simulink model "StopTrigger_Bench_2"  (R2025b)
settings: Solver=ode23t  StartTime=0.0  StopTime=3  MaxStep=1e-4  RelTol=1e-3
model workspace (MAT data in the model file):
  Ald = 5743.49177499
  GLDR = 1.5
  GPT = 1
  Ipk = 4.37e-06
  R1 = 10000
  Rfix = 10000
  Rhyst = 47000
  Rin = 1000
  Tend = 0.1
  Tstart = 1
  Ttrip = 0.5
  Vcc = 5
  VrefL = 3.82978723404
  VrefP = 2.9375
  gam = 0.8
  seedN = 1
  sigN = 0.01
  t0 = 1
  tau = 0.25
  tauL = 0.05
libraries: fl_lib x68, nesl_utility x24, ee_lib x11, simulink x5
(part 1 of 2)
settings Model: Creator=davin  LastModifiedBy=davin
settings DataIOCC: SaveOutput=off  ReturnWorkspaceOutputs=off

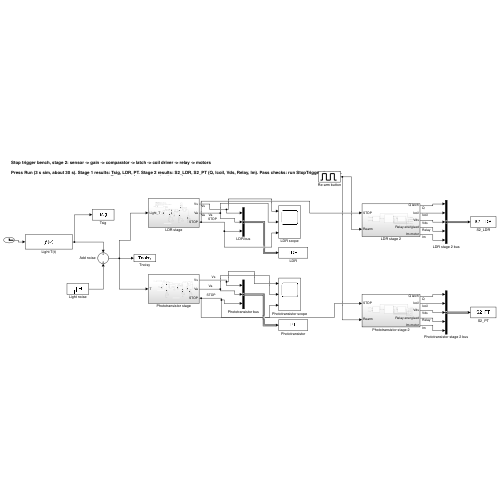
[thumbnail: Simulink's stored preview of the top-level diagram]
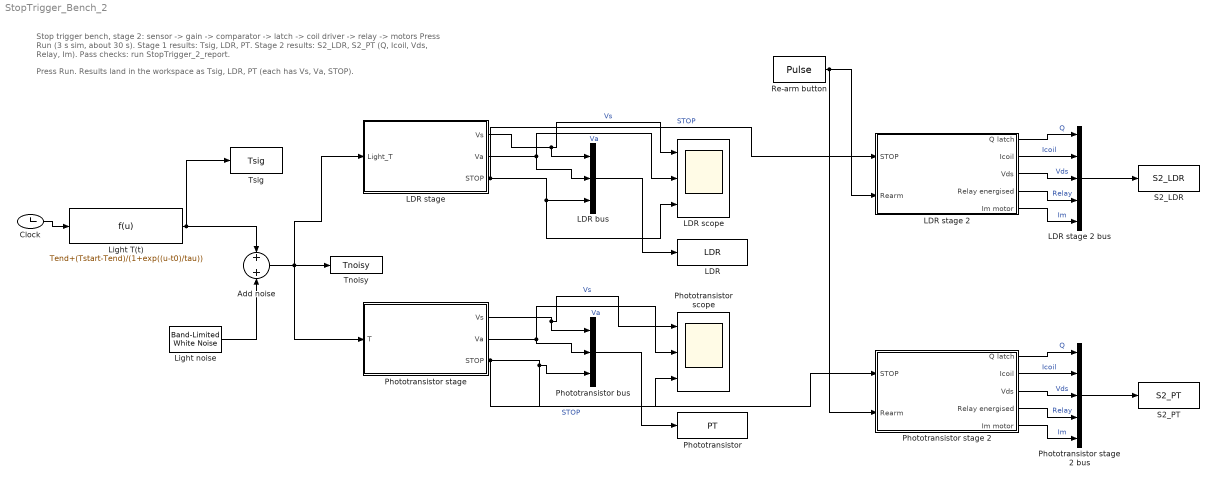
== system StopTrigger_Bench_2 ==
  note: Stop trigger bench, stage 2: sensor -> gain -> comparator -> latch -> coil driver -> relay -> motors
      |
      | Press Run (3 s sim, about 30 s). Stage 1 results: Tsig, LDR, PT. Stage 2 results: S2_LDR, S2_PT (Q, Icoil, Vds, Relay, Im). Pass checks: run StopTrigger_2_report.
  note: Press Run. Results land in the workspace as Tsig, LDR, PT (each has Vs, Va, STOP).
  Add noise : Sum
  Clock : Clock
  LDR : ToWorkspace  VariableName=LDR  SaveFormat=Timeseries  SampleTime=-1
  LDR bus : BusCreator  Inputs=3
  LDR scope : Scope  NumInputPorts=3
      settings: Title=Sensor node Vs (falls when dark)  ActiveDisplayYMinimum=0  ActiveDisplayYMaximum=5  YLabel=Vs [V]
  LDR stage : Subsystem
  LDR stage 2 : Subsystem
  LDR stage 2 bus : BusCreator  Inputs=5
  Light T(t) : Fcn  Expr=Tend+(Tstart-Tend)/(1+exp((u-t0)/tau))
  Light noise : simulink/Sources/Band-Limited White Noise  Cov=sigN^2*0.005  Ts=0.005  seed=[seedN]
  Phototransistor : ToWorkspace  VariableName=PT  SaveFormat=Timeseries  SampleTime=-1
  Phototransistor bus : BusCreator  Inputs=3
  Phototransistor scope : Scope  NumInputPorts=3
      settings: Title=Sensor node Vs (rises when dark)  ActiveDisplayYMinimum=0  ActiveDisplayYMaximum=5  YLabel=Vs [V]
  Phototransistor stage : Subsystem
  Phototransistor stage 2 : Subsystem
  Phototransistor stage 2 bus : BusCreator  Inputs=5
  Re-arm button : DiscretePulseGenerator  PulseType=Time based  Period=2.5  PulseWidth=2  SampleTime=0
  S2_LDR : ToWorkspace  VariableName=S2_LDR  SaveFormat=Timeseries  SampleTime=-1
  S2_PT : ToWorkspace  VariableName=S2_PT  SaveFormat=Timeseries  SampleTime=-1
  Tnoisy : ToWorkspace  VariableName=Tnoisy  SaveFormat=Timeseries  SampleTime=-1
  Tsig : ToWorkspace  VariableName=Tsig  SaveFormat=Timeseries  SampleTime=-1
  wires:
  Clock/1 -> Light T(t)/1
  LDR stage/1(Vs) -> LDR bus/1, LDR scope/1  "Vs"
  LDR stage/2(Va) -> LDR bus/2, LDR scope/2  "Va"
  LDR stage/3(STOP) -> LDR bus/3, LDR scope/3, LDR stage 2/1(STOP)  "STOP"
  LDR bus/1 -> LDR/1
  Phototransistor stage/1(Vs) -> Phototransistor bus/1, Phototransistor scope/1  "Vs"
  Phototransistor stage/2(Va) -> Phototransistor bus/2, Phototransistor scope/2  "Va"
  Phototransistor stage/3(STOP) -> Phototransistor bus/3, Phototransistor scope/3, Phototransistor stage 2/1(STOP)  "STOP"
  Phototransistor bus/1 -> Phototransistor/1
  Light T(t)/1 -> Add noise/1, Tsig/1
  Light noise/1 -> Add noise/2
  Add noise/1 -> LDR stage/1(Light_T), Tnoisy/1, Phototransistor stage/1(T)
  Re-arm button/1 -> LDR stage 2/2(Rearm), Phototransistor stage 2/2(Rearm)
  LDR stage 2/1(Q latch) -> LDR stage 2 bus/1  "Q"
  LDR stage 2/2(Icoil) -> LDR stage 2 bus/2  "Icoil"
  LDR stage 2/3(Vds) -> LDR stage 2 bus/3  "Vds"
  LDR stage 2/4(Relay energised) -> LDR stage 2 bus/4  "Relay"
  LDR stage 2/5(Im motor) -> LDR stage 2 bus/5  "Im"
  LDR stage 2 bus/1 -> S2_LDR/1
  Phototransistor stage 2/1(Q latch) -> Phototransistor stage 2 bus/1  "Q"
  Phototransistor stage 2/2(Icoil) -> Phototransistor stage 2 bus/2  "Icoil"
  Phototransistor stage 2/3(Vds) -> Phototransistor stage 2 bus/3  "Vds"
  Phototransistor stage 2/4(Relay energised) -> Phototransistor stage 2 bus/4  "Relay"
  Phototransistor stage 2/5(Im motor) -> Phototransistor stage 2 bus/5  "Im"
  Phototransistor stage 2 bus/1 -> S2_PT/1

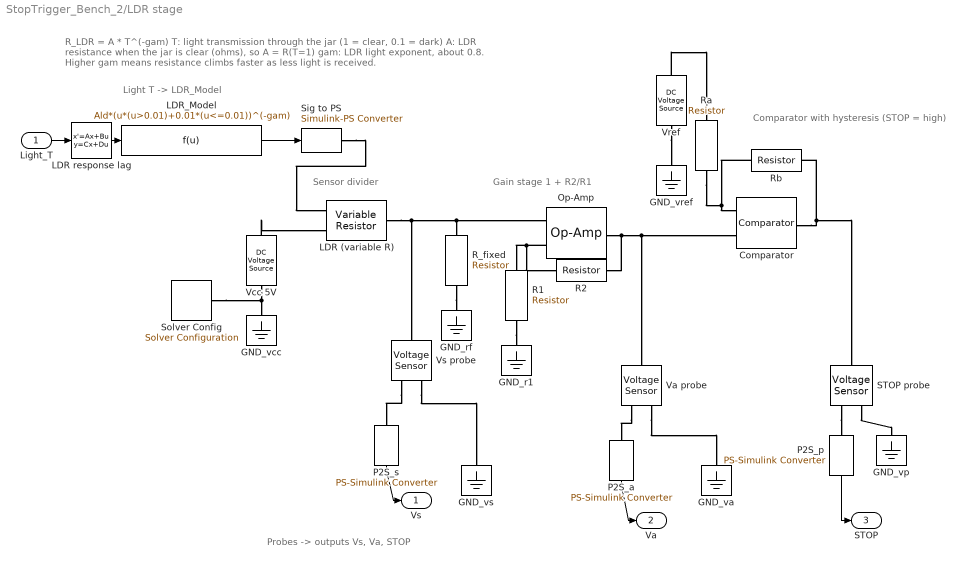
== system StopTrigger_Bench_2/LDR stage ==
  note: R_LDR = A * T^(-gam)
      |
      | T: light transmission through the jar (1 = clear, 0.1 = dark)
      |
      | A: LDR resistance when the jar is clear (ohms), so A = R(T=1)
      |
      | gam: LDR light exponent, about 0.8. Higher gam means resistance climbs faster as less light is received.
  note: Light T -> LDR_Model
  note: Sensor divider
  note: Gain stage 1 + R2/R1
  note: Comparator with hysteresis (STOP = high)
  note: Probes -> outputs Vs, Va, STOP
  Light_T : Inport
  Comparator : ee_lib/Integrated Circuits/Comparator  V_OS=5 mV  C_IN=0 pF  V_OL=0 V  V_OH=5 V  R_OUT=50 Ohm  Delay=0 s
      settings: InternalSimscapePortConfiguration="{\"Bottom\":[],\"Left\":[{\"id\":\"p\",\"label\":\"+\",\"type\":\"foundation.electrical.electrical\"},{\"id\":\"n\",\"label\":\"-\",\"type\":\"foundation.electrical.electrical\"}],\"Right\":[{\"id\":\"J\",\"label\":\"\",\"type\":\"foundation.electrical.electrical\"}],\"Top\":[]}"
  GND_r1 : fl_lib/Electrical/Electrical Elements/Electrical Reference
  GND_rf : fl_lib/Electrical/Electrical Elements/Electrical Reference
  GND_va : fl_lib/Electrical/Electrical Elements/Electrical Reference
  GND_vcc : fl_lib/Electrical/Electrical Elements/Electrical Reference
  GND_vp : fl_lib/Electrical/Electrical Elements/Electrical Reference
  GND_vref : fl_lib/Electrical/Electrical Elements/Electrical Reference
  GND_vs : fl_lib/Electrical/Electrical Elements/Electrical Reference
  LDR (variable R) : fl_lib/Electrical/Electrical Elements/Variable Resistor  Rmin=0 Ohm  thermalEnable=false  thermal_mass=1 J/K  i_specify=off  i_priority=None  i=0 A  i_nominal_specify=off  i_nominal_value=1  i_nominal_unit=A  v_specify=off  v_priority=None  v=0 V  v_nominal_specify=off  v_nominal_value=1  v_nominal_unit=V  T_specify=off  T_priority=None  T=300 K  T_nominal_specify=off  T_nominal_value=1  T_nominal_unit=K
  LDR response lag : StateSpace  A=-1/tauL  B=1/tauL  D=0  InitialCondition=Tstart
  LDR_Model : Fcn  Expr=Ald*(u*(u>0.01)+0.01*(u<=0.01))^(-gam)
  Op-Amp : fl_lib/Electrical/Electrical Elements/Op-Amp  outI_specify=off  outI_priority=None  outI=0 A  outI_nominal_specify=off  outI_nominal_value=1  outI_nominal_unit=A
  P2S_a : nesl_utility/PS-Simulink Converter  PhysicalDomain=network_engine_domain  SubClassName=ps_output  LeftPortType=input  RightPortType=output  PseudoPeriodic=off  Frequencies=[]  VectorFormat=inherit  Unit=inherit  AffineConversion=off
  P2S_p : nesl_utility/PS-Simulink Converter  PhysicalDomain=network_engine_domain  SubClassName=ps_output  LeftPortType=input  RightPortType=output  PseudoPeriodic=off  Frequencies=[]  VectorFormat=inherit  Unit=inherit  AffineConversion=off
  P2S_s : nesl_utility/PS-Simulink Converter  PhysicalDomain=network_engine_domain  SubClassName=ps_output  LeftPortType=input  RightPortType=output  PseudoPeriodic=off  Frequencies=[]  VectorFormat=inherit  Unit=inherit  AffineConversion=off
  R1 : fl_lib/Electrical/Electrical Elements/Resistor  R=R1 Ohm  i_specify=off  i_priority=None  i=0 A  i_nominal_specify=off  i_nominal_value=1  i_nominal_unit=A  v_specify=off  v_priority=None  v=0 V  v_nominal_specify=off  v_nominal_value=1  v_nominal_unit=V
  R2 : fl_lib/Electrical/Electrical Elements/Resistor  R=max((GLDR-1)*R1,1) Ohm  i_specify=off  i_priority=None  i=0 A  i_nominal_specify=off  i_nominal_value=1  i_nominal_unit=A  v_specify=off  v_priority=None  v=0 V  v_nominal_specify=off  v_nominal_value=1  v_nominal_unit=V
  R_fixed : fl_lib/Electrical/Electrical Elements/Resistor  R=Rfix Ohm  i_specify=off  i_priority=None  i=0 A  i_nominal_specify=off  i_nominal_value=1  i_nominal_unit=A  v_specify=off  v_priority=None  v=0 V  v_nominal_specify=off  v_nominal_value=1  v_nominal_unit=V
  Ra : fl_lib/Electrical/Electrical Elements/Resistor  R=Rin Ohm  i_specify=off  i_priority=None  i=0 A  i_nominal_specify=off  i_nominal_value=1  i_nominal_unit=A  v_specify=off  v_priority=None  v=0 V  v_nominal_specify=off  v_nominal_value=1  v_nominal_unit=V
  Rb : fl_lib/Electrical/Electrical Elements/Resistor  R=Rhyst Ohm  i_specify=off  i_priority=None  i=0 A  i_nominal_specify=off  i_nominal_value=1  i_nominal_unit=A  v_specify=off  v_priority=None  v=0 V  v_nominal_specify=off  v_nominal_value=1  v_nominal_unit=V
  STOP probe : fl_lib/Electrical/Electrical Sensors/Voltage Sensor
  Sig to PS : nesl_utility/Simulink-PS Converter  PhysicalDomain=network_engine_domain  SubClassName=ps_input  LeftPortType=input  RightPortType=output  PseudoPeriodic=off  Frequencies=[]  NoiseDistribution=none  NoiseParameters=[]  Unit=1  AffineConversion=off  FilteringAndDerivatives=provide  SimscapeFilterOrder=1  InputFilterTimeConstant=0.001  UdotUserProvided=0
  Solver Config : nesl_utility/Solver Configuration  PhysicalDomain=network_engine_domain  SubClassName=solver  LeftPortType=input  RightPortType=generic  Tones=[]  Harmonics=[]  SimulateNoise=off  Profile=off  UseLocalSampling=off  EnableSwitchedLinearOptims=on  FrequencyDomain=off  UseCCode=off  RelTol=0.001  AbsTol=0.001  MinStep=1e-09  ToWorkspace=off  RevertToSquareIcSolve=off  NumHomotopyIterations=100  PhasorMode=off  PhasorModeNumHarmonics=1  ConsistencySolver=NEWTON_XTOL_AFTER_FTOL  IndexReductionMethod=DerivativeReplacement  DoDC=off  ResidualTolerance=1e-09  ConsistencyTolSource=GLOBAL  ConsistencyAbsTol=0.001  ConsistencyRelTol=0.001  ConsistencyTolFactor=0.001  UseLocalSolver=off  LocalSolverChoice=NE_BACKWARD_EULER_ADVANCER  ResolveIndetEquations=on  FunctionEvalNumThread=1  LocalSolverSampleTime=0.001  DoFixedCost=off  MaxNonlinIter=3  MaxModeIter=2  ComputeImpulses=off  ImpulseIterations=2  LinearAlgebra=auto  LinearAlgebraNumThread=0  EquationFormulation=NE_TIME_EF  DelaysMemoryBudget=1024  AutomaticFiltering=on  FilteringTimeConstant=0.001  PartitionStorageMethod=AS_NEEDED  PartitionMemoryBudget=1024  PartitionMethod=ROBUST  MultibodyUseLocalSolver=off  MultibodyLocalSolverChoice=ODE1  MultibodyLocalSolverSampleTime=0.001
  Va probe : fl_lib/Electrical/Electrical Sensors/Voltage Sensor
  Vcc 5V : fl_lib/Electrical/Electrical Sources/DC Voltage Source  v0=Vcc V
  Vref : fl_lib/Electrical/Electrical Sources/DC Voltage Source  v0=VrefL V
  Vs probe : fl_lib/Electrical/Electrical Sensors/Voltage Sensor
  Vs : Outport
  Va : Outport  Port=2
  STOP : Outport  Port=3
  wires:
  LDR_Model/1 -> Sig to PS/1
  P2S_s/1 -> Vs/1
  P2S_a/1 -> Va/1
  P2S_p/1 -> STOP/1
  Light_T/1 -> LDR response lag/1
  LDR response lag/1 -> LDR_Model/1
  connections:
  Sig to PS/RConn1 -- LDR (variable R)/LConn1
  Vcc 5V/LConn1 -- LDR (variable R)/LConn2
  GND_vcc/LConn1 -- Vcc 5V/RConn1 -- Solver Config/RConn1
  R_fixed/LConn1 -- LDR (variable R)/RConn1 -- Vs probe/LConn1 -- Op-Amp/LConn1
  R_fixed/RConn1 -- GND_rf/LConn1
  Op-Amp/LConn2 -- R1/LConn1 -- R2/LConn1
  R1/RConn1 -- GND_r1/LConn1
  Op-Amp/RConn1 -- R2/RConn1 -- Va probe/LConn1 -- Comparator/LConn2
  Vref/LConn1 -- Ra/LConn1
  Vref/RConn1 -- GND_vref/LConn1
  Ra/RConn1 -- Rb/RConn1 -- Comparator/LConn1
  Rb/LConn1 -- STOP probe/LConn1 -- Comparator/RConn1
  Vs probe/RConn2 -- GND_vs/LConn1
  Va probe/RConn2 -- GND_va/LConn1
  STOP probe/RConn2 -- GND_vp/LConn1
  Vs probe/RConn1 -- P2S_s/LConn1
  Va probe/RConn1 -- P2S_a/LConn1
  STOP probe/RConn1 -- P2S_p/LConn1

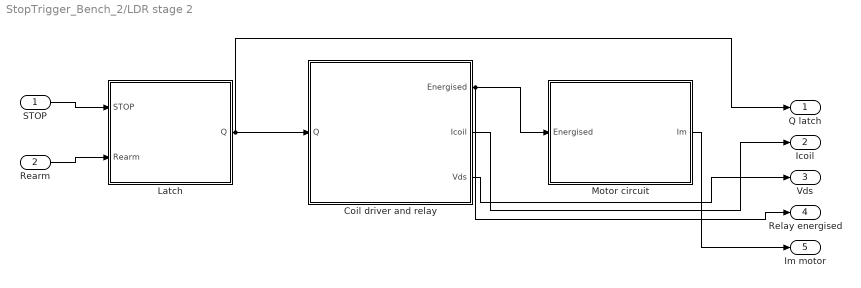
== system StopTrigger_Bench_2/LDR stage 2 ==
  STOP : Inport
  Rearm : Inport  Port=2
  Coil driver and relay : Subsystem
  Latch : Subsystem
  Motor circuit : Subsystem
  Q latch : Outport
  Icoil : Outport  Port=2
  Vds : Outport  Port=3
  Relay energised : Outport  Port=4
  Im motor : Outport  Port=5
  wires:
  STOP/1 -> Latch/1(STOP)
  Rearm/1 -> Latch/2(Rearm)
  Latch/1(Q) -> Coil driver and relay/1(Q), Q latch/1
  Coil driver and relay/2(Icoil) -> Icoil/1
  Coil driver and relay/1(Energised) -> Motor circuit/1(Energised), Relay energised/1
  Coil driver and relay/3(Vds) -> Vds/1
  Motor circuit/1(Im) -> Im motor/1

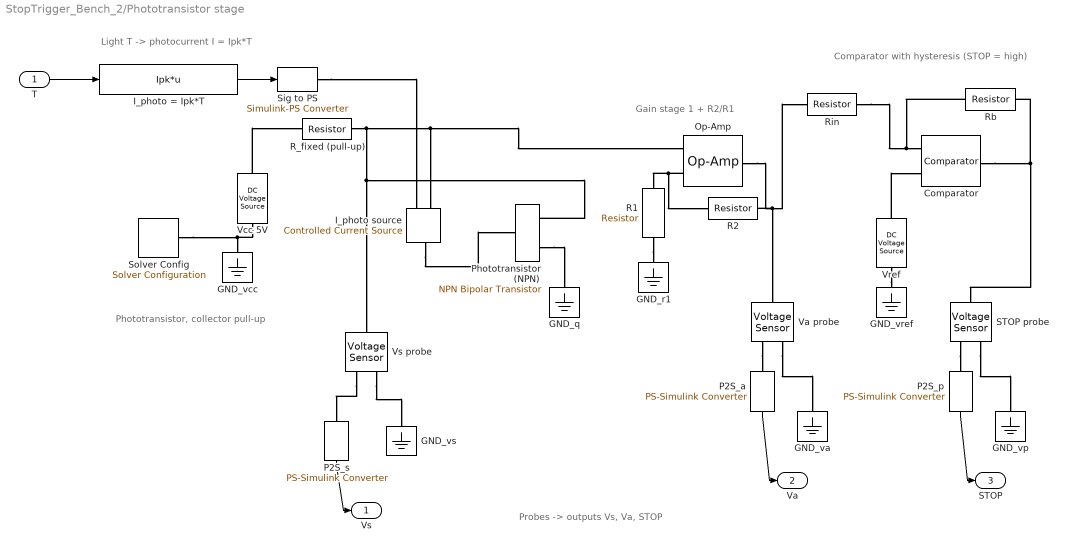
== system StopTrigger_Bench_2/Phototransistor stage ==
  note: Light T -> photocurrent I = Ipk*T
  note: Phototransistor, collector pull-up
  note: Gain stage 1 + R2/R1
  note: Comparator with hysteresis (STOP = high)
  note: Probes -> outputs Vs, Va, STOP
  T : Inport
  Comparator : ee_lib/Integrated Circuits/Comparator  V_OS=5 mV  C_IN=0 pF  V_OL=0 V  V_OH=5 V  R_OUT=50 Ohm  Delay=0 s
      settings: InternalSimscapePortConfiguration="{\"Bottom\":[],\"Left\":[{\"id\":\"p\",\"label\":\"+\",\"type\":\"foundation.electrical.electrical\"},{\"id\":\"n\",\"label\":\"-\",\"type\":\"foundation.electrical.electrical\"}],\"Right\":[{\"id\":\"J\",\"label\":\"\",\"type\":\"foundation.electrical.electrical\"}],\"Top\":[]}"
  GND_q : fl_lib/Electrical/Electrical Elements/Electrical Reference
  GND_r1 : fl_lib/Electrical/Electrical Elements/Electrical Reference
  GND_va : fl_lib/Electrical/Electrical Elements/Electrical Reference
  GND_vcc : fl_lib/Electrical/Electrical Elements/Electrical Reference
  GND_vp : fl_lib/Electrical/Electrical Elements/Electrical Reference
  GND_vref : fl_lib/Electrical/Electrical Elements/Electrical Reference
  GND_vs : fl_lib/Electrical/Electrical Elements/Electrical Reference
  I_photo = Ipk*T : Fcn  Expr=Ipk*u
  I_photo source : fl_lib/Electrical/Electrical Sources/Controlled Current Source
  Op-Amp : fl_lib/Electrical/Electrical Elements/Op-Amp  outI_specify=off  outI_priority=None  outI=0 A  outI_nominal_specify=off  outI_nominal_value=1  outI_nominal_unit=A
  P2S_a : nesl_utility/PS-Simulink Converter  PhysicalDomain=network_engine_domain  SubClassName=ps_output  LeftPortType=input  RightPortType=output  PseudoPeriodic=off  Frequencies=[]  VectorFormat=inherit  Unit=inherit  AffineConversion=off
  P2S_p : nesl_utility/PS-Simulink Converter  PhysicalDomain=network_engine_domain  SubClassName=ps_output  LeftPortType=input  RightPortType=output  PseudoPeriodic=off  Frequencies=[]  VectorFormat=inherit  Unit=inherit  AffineConversion=off
  P2S_s : nesl_utility/PS-Simulink Converter  PhysicalDomain=network_engine_domain  SubClassName=ps_output  LeftPortType=input  RightPortType=output  PseudoPeriodic=off  Frequencies=[]  VectorFormat=inherit  Unit=inherit  AffineConversion=off
  Phototransistor (NPN) : ee_lib/Semiconductors & Converters/NPN Bipolar Transistor  parameterization=1  BF=100  IS=1e-14 A  VAF=200 V  hfe=100  hoe=50e-6 1/Ohm  Ic_h=1 mA  Vce_h=5 V  V1=0.55 V  I1=0.5 mA  BR=1  Tmeas=25 degC  RC=0.01 Ohm  RE=1e-4 Ohm  RB=1 Ohm  C_BC=5 pF  C_BE=5 pF  TF=0 us  TR=0 us  prmDatasheet=1  prmEquCoeff=1  hfe_T2=125  XTB=0  V1_T2=0.45 V  I1_T2=0.5 mA  Tmeas2=125 degC  EG=1.11 eV  XTI=3  TdeviceDatasheet=25 degC  TdeviceEquCoeff=25 degC  ec=1  ib_specify=off  ib_priority=None  ib=0 A  ib_nominal_specify=off  ib_nominal_value=1  ib_nominal_unit=A  ic_specify=off  ic_priority=None  ic=0 A  ic_nominal_specify=off  ic_nominal_value=1  ic_nominal_unit=A  vce_specify=off  vce_priority=None  vce=0 V  vce_nominal_specify=off  vce_nominal_value=1  vce_nominal_unit=V  vbe_specify=off  vbe_priority=None  vbe=0 V  vbe_nominal_specify=off  vbe_nominal_value=1  vbe_nominal_unit=V  Qbc_specify=off  Qbc_priority=High  Qbc=0 C  Qbc_nominal_specify=off  Qbc_nominal_value=1  Qbc_nominal_unit=uC  Qbe_specify=off  Qbe_priority=High  Qbe=0 C  Qbe_nominal_specify=off  Qbe_nominal_value=1  Qbe_nominal_unit=uC  thermal_network_parameterization=ee.enum.thermalNetworkTopology.junctionCase  Rth=[0, 10] K/W  Rth_Cauer=[1, 3, 10] K/W  Rth_Foster=[.08, .14, .22, .16] K/W  thermal_mass_parameterization=ee.enum.thermalNetwork.timeconstant  thermal_mass=[0, 1] J/K  thermal_mass_Cauer=[.1, .3, 1] J/K  thermal_mass_Foster=[.001, .005, .05, .5] J/K  thermal_time_constant=[0, 10] s  thermal_time_constant_Cauer=[1, 3, 10] s  thermal_time_constant_Foster=[7e-05, .0007, .01, .08] s  thermal_mass_initial_temperatures=[25, 25] degC  thermal_mass_initial_temperatures_Cauer=[25, 25, 25] degC  Tvec_initial_Foster=[25, 25, 25, 25] degC
      settings: InternalSimscapePortConfiguration="{\"Bottom\":[],\"Left\":[{\"id\":\"B\",\"label\":\"\",\"type\":\"foundation.electrical.electrical\"}],\"Right\":[{\"id\":\"C\",\"label\":\"\",\"type\":\"foundation.electrical.electrical\"},{\"id\":\"E\",\"label\":\"\",\"type\":\"foundation.electrical.electrical\"}],\"Top\":[]}"
  R1 : fl_lib/Electrical/Electrical Elements/Resistor  R=R1 Ohm  i_specify=off  i_priority=None  i=0 A  i_nominal_specify=off  i_nominal_value=1  i_nominal_unit=A  v_specify=off  v_priority=None  v=0 V  v_nominal_specify=off  v_nominal_value=1  v_nominal_unit=V
  R2 : fl_lib/Electrical/Electrical Elements/Resistor  R=max((GPT-1)*R1,1) Ohm  i_specify=off  i_priority=None  i=0 A  i_nominal_specify=off  i_nominal_value=1  i_nominal_unit=A  v_specify=off  v_priority=None  v=0 V  v_nominal_specify=off  v_nominal_value=1  v_nominal_unit=V
  R_fixed (pull-up) : fl_lib/Electrical/Electrical Elements/Resistor  R=Rfix Ohm  i_specify=off  i_priority=None  i=0 A  i_nominal_specify=off  i_nominal_value=1  i_nominal_unit=A  v_specify=off  v_priority=None  v=0 V  v_nominal_specify=off  v_nominal_value=1  v_nominal_unit=V
  Rb : fl_lib/Electrical/Electrical Elements/Resistor  R=Rhyst Ohm  i_specify=off  i_priority=None  i=0 A  i_nominal_specify=off  i_nominal_value=1  i_nominal_unit=A  v_specify=off  v_priority=None  v=0 V  v_nominal_specify=off  v_nominal_value=1  v_nominal_unit=V
  Rin : fl_lib/Electrical/Electrical Elements/Resistor  R=Rin Ohm  i_specify=off  i_priority=None  i=0 A  i_nominal_specify=off  i_nominal_value=1  i_nominal_unit=A  v_specify=off  v_priority=None  v=0 V  v_nominal_specify=off  v_nominal_value=1  v_nominal_unit=V
  STOP probe : fl_lib/Electrical/Electrical Sensors/Voltage Sensor
  Sig to PS : nesl_utility/Simulink-PS Converter  PhysicalDomain=network_engine_domain  SubClassName=ps_input  LeftPortType=input  RightPortType=output  PseudoPeriodic=off  Frequencies=[]  NoiseDistribution=none  NoiseParameters=[]  Unit=1  AffineConversion=off  FilteringAndDerivatives=provide  SimscapeFilterOrder=1  InputFilterTimeConstant=0.001  UdotUserProvided=0
  Solver Config : nesl_utility/Solver Configuration  PhysicalDomain=network_engine_domain  SubClassName=solver  LeftPortType=input  RightPortType=generic  Tones=[]  Harmonics=[]  SimulateNoise=off  Profile=off  UseLocalSampling=off  EnableSwitchedLinearOptims=on  FrequencyDomain=off  UseCCode=off  RelTol=0.001  AbsTol=0.001  MinStep=1e-09  ToWorkspace=off  RevertToSquareIcSolve=off  NumHomotopyIterations=100  PhasorMode=off  PhasorModeNumHarmonics=1  ConsistencySolver=NEWTON_XTOL_AFTER_FTOL  IndexReductionMethod=DerivativeReplacement  DoDC=off  ResidualTolerance=1e-09  ConsistencyTolSource=GLOBAL  ConsistencyAbsTol=0.001  ConsistencyRelTol=0.001  ConsistencyTolFactor=0.001  UseLocalSolver=off  LocalSolverChoice=NE_BACKWARD_EULER_ADVANCER  ResolveIndetEquations=on  FunctionEvalNumThread=1  LocalSolverSampleTime=0.001  DoFixedCost=off  MaxNonlinIter=3  MaxModeIter=2  ComputeImpulses=off  ImpulseIterations=2  LinearAlgebra=auto  LinearAlgebraNumThread=0  EquationFormulation=NE_TIME_EF  DelaysMemoryBudget=1024  AutomaticFiltering=on  FilteringTimeConstant=0.001  PartitionStorageMethod=AS_NEEDED  PartitionMemoryBudget=1024  PartitionMethod=ROBUST  MultibodyUseLocalSolver=off  MultibodyLocalSolverChoice=ODE1  MultibodyLocalSolverSampleTime=0.001
  Va probe : fl_lib/Electrical/Electrical Sensors/Voltage Sensor
  Vcc 5V : fl_lib/Electrical/Electrical Sources/DC Voltage Source  v0=Vcc V
  Vref : fl_lib/Electrical/Electrical Sources/DC Voltage Source  v0=VrefP V
  Vs probe : fl_lib/Electrical/Electrical Sensors/Voltage Sensor
  Vs : Outport
  Va : Outport  Port=2
  STOP : Outport  Port=3
  wires:
  T/1 -> I_photo = Ipk*T/1
  I_photo = Ipk*T/1 -> Sig to PS/1
  P2S_s/1 -> Vs/1
  P2S_a/1 -> Va/1
  P2S_p/1 -> STOP/1
  connections:
  Sig to PS/RConn1 -- I_photo source/RConn1
  Vcc 5V/LConn1 -- R_fixed (pull-up)/LConn1
  GND_vcc/LConn1 -- Vcc 5V/RConn1 -- Solver Config/RConn1
  Phototransistor (NPN)/RConn1 -- Op-Amp/LConn1 -- I_photo source/RConn2 -- R_fixed (pull-up)/RConn1 -- Vs probe/LConn1
  I_photo source/LConn1 -- Phototransistor (NPN)/LConn1
  Phototransistor (NPN)/RConn2 -- GND_q/LConn1
  R1/LConn1 -- Op-Amp/LConn2 -- R2/LConn1
  R1/RConn1 -- GND_r1/LConn1
  R2/RConn1 -- Op-Amp/RConn1 -- Rin/LConn1 -- Va probe/LConn1
  Comparator/LConn1 -- Rin/RConn1 -- Rb/RConn1
  Comparator/RConn1 -- Rb/LConn1 -- STOP probe/LConn1
  Vref/LConn1 -- Comparator/LConn2
  Vref/RConn1 -- GND_vref/LConn1
  Vs probe/RConn2 -- GND_vs/LConn1
  Va probe/RConn2 -- GND_va/LConn1
  STOP probe/RConn2 -- GND_vp/LConn1
  Vs probe/RConn1 -- P2S_s/LConn1
  Va probe/RConn1 -- P2S_a/LConn1
  STOP probe/RConn1 -- P2S_p/LConn1

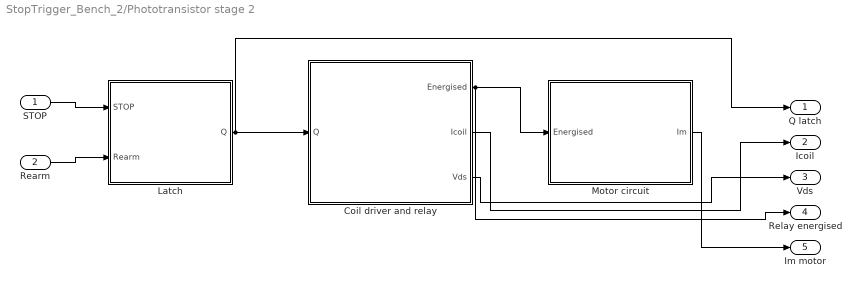
== system StopTrigger_Bench_2/Phototransistor stage 2 ==
  STOP : Inport
  Rearm : Inport  Port=2
  Coil driver and relay : Subsystem
  Latch : Subsystem
  Motor circuit : Subsystem
  Q latch : Outport
  Icoil : Outport  Port=2
  Vds : Outport  Port=3
  Relay energised : Outport  Port=4
  Im motor : Outport  Port=5
  wires:
  Motor circuit/1(Im) -> Im motor/1
  Coil driver and relay/3(Vds) -> Vds/1
  Coil driver and relay/1(Energised) -> Relay energised/1, Motor circuit/1(Energised)
  Coil driver and relay/2(Icoil) -> Icoil/1
  Latch/1(Q) -> Q latch/1, Coil driver and relay/1(Q)
  Rearm/1 -> Latch/2(Rearm)
  STOP/1 -> Latch/1(STOP)

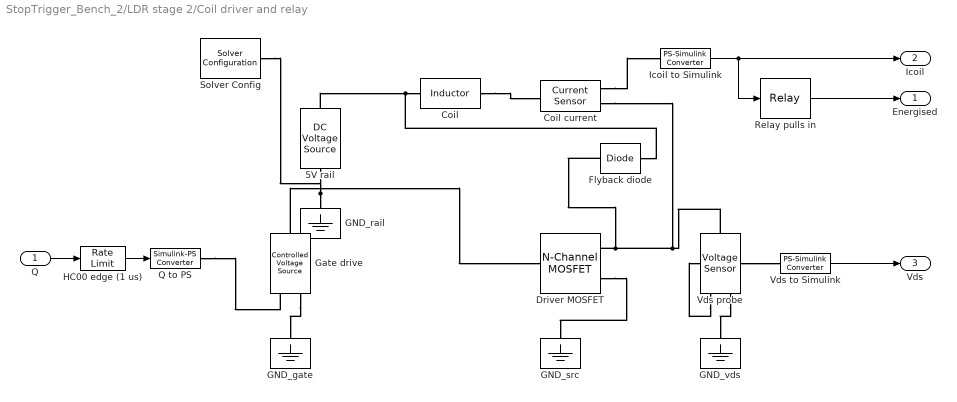
== system StopTrigger_Bench_2/LDR stage 2/Coil driver and relay ==
  Q : Inport
  5V rail : fl_lib/Electrical/Electrical Sources/DC Voltage Source  v0=5 V
  Coil : fl_lib/Electrical/Electrical Elements/Inductor  l=0.1 H  r=63.3 Ohm  g=1e-9 1/Ohm  i_specify=off  i_priority=None  i=0 A  i_nominal_specify=off  i_nominal_value=1  i_nominal_unit=A  v_specify=off  v_priority=None  v=0 V  v_nominal_specify=off  v_nominal_value=1  v_nominal_unit=V  i_L_specify=off  i_L_priority=High  i_L=0 A  i_L_nominal_specify=off  i_L_nominal_value=1  i_L_nominal_unit=A
  Coil current : fl_lib/Electrical/Electrical Sensors/Current Sensor
  Driver MOSFET : ee_lib/Semiconductors & Converters/N-Channel MOSFET  paramTerminal=ee.enum.mosfet.numberOfTerminals.three  parameterization=ee.enum.mosfet.parameterization.datasheet  Beta=5.0 A/V^2  Rds=0.022 Ohm  Id=25 A  Vgs=5 V  Vth=1.7 V  Vth0=1.7 V  lam=0 1/V  gamma_vth=0.5 V^(1/2)  phib=0.5 V  Vth1=1.9071 V  Vbs1=-1 V  Vth2=2.066 V  Vbs2=-2 V  Tmeas=25 degC  Vgs_vec=[-1, -.5, 2, 3, 4, 5] V  Vds_vec=[0, 2, 4, 8, 12, 16, 20] V  Vbs_vec=[0, -4, -6, -12] V  T_vec=[25, 125] degC  Vth_vec=[.4, 1.2, 1.4, 1.45] V  Vth_mat=[.4, .35; 1.2, 1.15; 1.4, 1.35; 1.45, 1.4] V  Ids_mat=[0, 0, 0, 0, 0, 0, 0; 0, 0, 0, 0, 0, 0, 0; 0, .003, .0038, .0043, .0046, .0048, .0049; 0, .0055, .008, .009, .0095, .01, .0101; 0, .0115, .016, .018, .019, .0195, .02; 0, .0152, .0225, .0265, .028, .0295, .03] A  Ids_mat0=[0, 0, 0, 0, 0, 0, 0; 0, 0, 0, 0, 0, 0, 0; 0, .003, .0038, .0043, .0046, .0048, .0049; 0, .0055, .008, .009, .0095, .01, .0101; 0, .0115, .016, .018, .019, .0195, .02; 0, .0152, .0225, .0265, .028, .0295, .03] A  Ids_mat_3D=zeros(6, 7, 2) A  Ids_mat_3D0=zeros(6, 7, 2) A  IV_table_symmetry=ee.enum.mosfet.symmetricNIV.no  RS=0.0001 Ohm  RD=0.01 Ohm  RB=0.001 Ohm  LeadRs=0 Ohm  LeadRd=0 Ohm  LeadRg=0 Ohm  LeadRb=0 Ohm  LS=0 nH  LD=0 nH  LG=0 nH  LB=0 nH  C_param=ee.enum.mosfet.capacitanceParam.fixedciss  C_GS=270 pF  C_GD=80 pF  C_GB=0 pF  C_DS=0 pF  C_iss=350 pF  C_rss=80 pF  C_oss=0 pF  C_iss_vec=[720, 700, 590, 470, 390, 310] pF  C_rss_vec=[450, 400, 300, 190, 95, 55] pF  C_oss_vec=[900, 810, 690, 420, 270, 170] pF  C_GS_vec=[270, 300, 290, 280, 295, 255] pF  C_GD_vec=[450, 400, 300, 190, 95, 55] pF  C_GB_vec=[270, 300, 290, 280, 295, 255] pF  C_Vgs_vec=0 V  C_DS_vec=[450, 410, 390, 230, 175, 115] pF  C_Vds_vec=[.1, .3, 1, 3, 10, 30] V  V_GS_for_cap_data=0 V  charge_linearity_param=ee.enum.mosfet.cgdLinearity.constant  C_OX=200 pF  V_C_OX=-0.5 V  charge_linearity_param_vgb=ee.enum.mosfet.cgbLinearity.instantly  charge_linearity_param_with_vgb=ee.enum.mosfet.cgbLinearityWithSeparateCgb.instantly  Di_param=ee.enum.mosfet.diodeParam.no  IsDiode=1e-12 A  Vbi=0.6 V  n=1  Cj0Diode=0 pF  TT=50e-9 s  Tmeas_dio=25 degC  TableTypeNoT=ee.enum.mosfet.tableType.IfMat  TableType=ee.enum.diode.tableType.IfMat  IfVec=[.07, .12, .19, 1.75, 4.24, 7.32, 11.2] A  IfMat=[.07, .12, .19, 1.75, 4.24, 7.32, 11.2; .16, .3, .72, 2.14, 4.02, 6.35, 9.12] A  VfVecV=[.9, 1.15, 1.25, 1.5, 1.75, 2.17, 2.6, 2.85] V  VfMatV=[.9, 1.15, 1.25, 1.5, 1.75, 2.17, 2.6, 2.85; .58, .68, .75, 1.1, 1.38, 1.77, 2.27, 2.7] V  TjVec=[25, 125] degC  VfVec=[.5, .7, .9, 1.3, 1.7, 2.1, 2.5] V  IfVecV=[.1, .2, .5, 1, 2, 4, 7, 10] A  diode_Goff=1e-12 1/Ohm  prmDatasheet=ee.enum.temperatureParameterization.none  prmEquCoeff=ee.enum.temperatureParameterization.none  dVth_dT=-6 mV/K  dVth0_dT=-6 mV/K  Rds_T2=0.037 Ohm  BEXDatasheet=-1.5  BEXEquCoeff=-1.5  etaisDatasheet=3  etaisEquCoeff=3  Tmeas2=125 degC  etaisTabulated=3  TdeviceDatasheet=25 degC  TdeviceEquCoeff=25 degC  TdeviceTabulated=25 degC  i_g_specify=off  i_g_priority=None  i_g=0 A  i_g_nominal_specify=off  i_g_nominal_value=1  i_g_nominal_unit=A  i_d_specify=off  i_d_priority=None  i_d=0 A  i_d_nominal_specify=off  i_d_nominal_value=1  i_d_nominal_unit=A  i_b_specify=off  i_b_priority=None  i_b=0 A  i_b_nominal_specify=off  i_b_nominal_value=1  i_b_nominal_unit=A  voltage_gs_specify=off  voltage_gs_priority=None  voltage_gs=0 V  voltage_gs_nominal_specify=off  voltage_gs_nominal_value=1  voltage_gs_nominal_unit=V  voltage_ds_specify=off  voltage_ds_priority=None  voltage_ds=0 V  voltage_ds_nominal_specify=off  voltage_ds_nominal_value=1  voltage_ds_nominal_unit=V  voltage_bs_specify=off  voltage_bs_priority=None  voltage_bs=0 V  voltage_bs_nominal_specify=off  voltage_bs_nominal_value=1  voltage_bs_nominal_unit=V  v_Cgs_specify=off  v_Cgs_priority=High  v_Cgs=0 V  v_Cgs_nominal_specify=off  v_Cgs_nominal_value=1  v_Cgs_nominal_unit=V  v_Cds_specify=off  v_Cds_priority=High  v_Cds=0 V  v_Cds_nominal_specify=off  v_Cds_nominal_value=1  v_Cds_nominal_unit=V  v_Cbs_specify=off  v_Cbs_priority=High  v_Cbs=0 V  v_Cbs_nominal_specify=off  v_Cbs_nominal_value=1  v_Cbs_nominal_unit=V  thermal_network_parameterization=ee.enum.thermalNetworkTopology.junctionCase  Rth=[0, 10] K/W  Rth_Cauer=[1, 3, 10] K/W  Rth_Foster=[.08, .14, .22, .16] K/W  thermal_mass_parameterization=ee.enum.thermalNetwork.timeconstant  thermal_mass=[0, 1] J/K  thermal_mass_Cauer=[.1, .3, 1] J/K  thermal_mass_Foster=[.001, .005, .05, .5] J/K  thermal_time_constant=[0, 10] s  thermal_time_constant_Cauer=[1, 3, 10] s  thermal_time_constant_Foster=[7e-05, .0007, .01, .08] s  thermal_mass_initial_temperatures=[25, 25] degC  thermal_mass_initial_temperatures_Cauer=[25, 25, 25] degC  Tvec_initial_Foster=[25, 25, 25, 25] degC  betaref=18 A/V^2  Vfbref=-1.1 V  gamma=3.5 V^(1/2)  phib2ref=1 V  thesatref=0.4 1/V  alpha=0  Vp=5e-2 V  thesrref=0 1/V  m=8  Tref=25 degC  Rsref=2e-3 Ohm  Rdref=0.17 Ohm  Rgref=8.4 Ohm  Rbref=2e-3 Ohm  Cox=1500 pF  Cgso=100 pF  Cgdo=14 pF  Isref=5.2e-13 A  Cj0=480 pF  Tprm=1  etabet=1.3  Stvfb=5e-4 V/K  Stphib=-8.5e-4 V/K  etasat=1.04  etasr=0.65  etar=0.95  etais=3  Tsim=25 degC  Ig_specify=off  Ig_priority=None  Ig=0 A  Ig_nominal_specify=off  Ig_nominal_value=1  Ig_nominal_unit=nA  Ids_specify=off  Ids_priority=None  Ids=0 A  Ids_nominal_specify=off  Ids_nominal_value=1  Ids_nominal_unit=A  Ib_specify=off  Ib_priority=None  Ib=0 A  Ib_nominal_specify=off  Ib_nominal_value=1  Ib_nominal_unit=uA  V_gs_specify=off  V_gs_priority=None  V_gs=0 V  V_gs_nominal_specify=off  V_gs_nominal_value=1  V_gs_nominal_unit=V  V_ds_specify=off  V_ds_priority=None  V_ds=0 V  V_ds_nominal_specify=off  V_ds_nominal_value=1  V_ds_nominal_unit=V  V_bs_specify=off  V_bs_priority=None  V_bs=0 V  V_bs_nominal_specify=off  V_bs_nominal_value=1  V_bs_nominal_unit=V  QGoverCox_specify=off  QGoverCox_priority=None  QGoverCox=0 V  QGoverCox_nominal_specify=off  QGoverCox_nominal_value=1  QGoverCox_nominal_unit=V  QDoverCox_specify=off  QDoverCox_priority=None  QDoverCox=0 V  QDoverCox_nominal_specify=off  QDoverCox_nominal_value=1  QDoverCox_nominal_unit=V  QBoverCox_specify=off  QBoverCox_priority=None  QBoverCox=0 V  QBoverCox_nominal_specify=off  QBoverCox_nominal_value=1  QBoverCox_nominal_unit=V  T0=[25, 25] degC  T0_Cauer=[25, 25, 25] degC
  Flyback diode : ee_lib/Semiconductors & Converters/Diode  ModelType=ee.enum.diode.modelType.pwl  TableType=ee.enum.diode.tableType.IfMat  IfMat=[.07, .12, .19, 1.75, 4.24, 7.32, 11.2; .16, .3, .72, 2.14, 5.02, 8.35, 13.12] A  VfMat=[.9, 1.15, 1.25, 1.5, 1.75, 2.17, 2.6, 2.85; .58, .68, .75, 1.1, 1.38, 1.77, 2.27, 2.7] V  TjVec=[25, 125] degC  VfVec=[.5, .7, .9, 1.3, 1.7, 2.1, 2.5] V  IfVec=[.1, .2, .5, 1, 2, 4, 7, 10] A  IrMat=[1e-06, 2e-06, 5e-06, 1e-05, 2.5e-05, 5e-05, .0001; 2e-06, 5e-06, 1e-05, 4e-05, 8e-05, .0002, .0005] A  VrMat=[10, 100, 200, 250, 300, 325, 350; 10, 70, 160, 220, 270, 300, 320] V  VrVec=[10, 20, 40, 50, 70, 80, 100] V  IrVec=[1e-06, 2e-06, 5e-06, 1e-05, 2e-05, 5e-05, .0001] A  Vf=0.6 V  Ron=0.3 Ohm  Goff=1e-8 S  prmExp=ee.enum.diode.expParam.useTwo  I12=[.0137, .545] A  V12=[.6, .7] V  RS=0 Ohm  Tmeas=298.15 K  IS=1e-12 A  ec=1  I1=0.0137 A  V1=0.6 V  N_series=1  N_parallel=1  ZenerEnable=false  Rz=0.3 Ohm  BV=inf V  C_param=ee.enum.diode.capParam.fixed  CJ=0 pF  CJ0=5 pF  Vvec=[.1, 10, 100] V  Cvec=[3.5, 1, .4] pF  VJ=1 V  Mgrad=0.5  FC=0.5  Q_param=ee.enum.diode.recoveryParam.off  iRM=-7.15 A  iF=4 A  didt=-750 A/us  trr_factor=3  trr=115 ns  Qrr=150 nA*s  Vr=-600 V  Ls=150 nH  Erec=0.03 J  TT=50 ns  tau=100 ns  T_param=ee.enum.diode.temperatureParam.off  Tdevice=298.15 K  I1_T2=0.245 A  V1_T2=0.5 V  IS_T2=1.25e-7 A  Tmeas2=125 degC  XTI_param=ee.enum.diode.xtiParam.pn  XTI=3  EG_param=ee.enum.diode.egapParam.material_si  EG=1.11 eV  dBVdT=0 V/K  enable_fault_input=simscape.enum.onoff.off  i_specify=off  i_priority=None  i=0 A  i_nominal_specify=off  i_nominal_value=1  i_nominal_unit=A  v_specify=off  v_priority=None  v=0 V  v_nominal_specify=off  v_nominal_value=1  v_nominal_unit=V  v_capacitor_specify=off  v_capacitor_priority=None  v_capacitor=0 V  v_capacitor_nominal_specify=off  v_capacitor_nominal_value=1  v_capacitor_nominal_unit=V  Qj_specify=off  Qj_priority=High  Qj=0 C  Qj_nominal_specify=off  Qj_nominal_value=1  Qj_nominal_unit=C  i_diode_specify=off  i_diode_priority=None  i_diode=0 A  i_diode_nominal_specify=off  i_diode_nominal_value=1  i_diode_nominal_unit=A  v_diode_specify=off  v_diode_priority=None  v_diode=0 V  v_diode_nominal_specify=off  v_diode_nominal_value=1  v_diode_nominal_unit=V  i_capacitor_specify=off  i_capacitor_priority=None  i_capacitor=0 A  i_capacitor_nominal_specify=off  i_capacitor_nominal_value=1  i_capacitor_nominal_unit=A  power_dissipated_specify=off  power_dissipated_priority=None  power_dissipated=0 W  power_dissipated_nominal_specify=off  power_dissipated_nominal_value=1  power_dissipated_nominal_unit=W  fidelity_level=ee.enum.diode.fidelity.includeChargeDyn  rec_loss_model=ee.enum.diode.reverseRecoveryModel.fixed  ErecVal=0 J  scaleWithIandV=true  ErecMat=zeros(2, 3) J  TjrecVec=[298.15, 398.15] K  IfrecVec=[.1, 1, 10] A  IrecVal=10 A  VrecVal=10 V  tFilter=1 / 1000 / 100 s  thermal_network_parameterization=ee.enum.thermalNetworkTopology.junctionCase  Rth=[0, 10] K/W  Rth_Cauer=[1, 3, 10] K/W  Rth_Foster=[.08, .14, .22, .16] K/W  thermal_mass_parameterization=ee.enum.thermalNetwork.timeconstant  thermal_mass=[0, 1] J/K  thermal_mass_Cauer=[.1, .3, 1] J/K  thermal_mass_Foster=[.001, .005, .05, .5] J/K  thermal_time_constant=[0, 10] s  thermal_time_constant_Cauer=[1, 3, 10] s  thermal_time_constant_Foster=[7e-05, .0007, .01, .08] s  thermal_mass_initial_temperatures=[25, 25] degC  thermal_mass_initial_temperatures_Cauer=[25, 25, 25] degC  junction_thermal_mass=0.01 J/K  Tvec_initial_Foster=[25, 25, 25, 25] degC  no_thermal_network=0  junction_temperature_specify=off  junction_temperature_priority=None  junction_temperature=25 degC  junction_temperature_nominal_specify=off  junction_temperature_nominal_value=1  junction_temperature_nominal_unit=degC
  GND_gate : fl_lib/Electrical/Electrical Elements/Electrical Reference
  GND_rail : fl_lib/Electrical/Electrical Elements/Electrical Reference
  GND_src : fl_lib/Electrical/Electrical Elements/Electrical Reference
  GND_vds : fl_lib/Electrical/Electrical Elements/Electrical Reference
  Gate drive : fl_lib/Electrical/Electrical Sources/Controlled Voltage Source
  HC00 edge (1 us) : RateLimiter  RisingSlewLimit=5e6  FallingSlewLimit=-5e6  SampleTimeMode=inherited
  Icoil to Simulink : nesl_utility/PS-Simulink Converter  PhysicalDomain=network_engine_domain  SubClassName=ps_output  LeftPortType=input  RightPortType=output  PseudoPeriodic=off  Frequencies=[]  VectorFormat=inherit  Unit=inherit  AffineConversion=off
  Q to PS : nesl_utility/Simulink-PS Converter  PhysicalDomain=network_engine_domain  SubClassName=ps_input  LeftPortType=input  RightPortType=output  PseudoPeriodic=off  Frequencies=[]  NoiseDistribution=none  NoiseParameters=[]  Unit=1  AffineConversion=off  FilteringAndDerivatives=filter  SimscapeFilterOrder=1  InputFilterTimeConstant=1e-6  UdotUserProvided=0
  Relay pulls in : Relay  OnSwitchValue=0.0593  OffSwitchValue=0.0079
  Solver Config : nesl_utility/Solver Configuration  PhysicalDomain=network_engine_domain  SubClassName=solver  LeftPortType=input  RightPortType=generic  Tones=[]  Harmonics=[]  SimulateNoise=off  Profile=off  UseLocalSampling=off  EnableSwitchedLinearOptims=on  FrequencyDomain=off  UseCCode=off  RelTol=0.001  AbsTol=0.001  MinStep=1e-09  ToWorkspace=off  RevertToSquareIcSolve=off  NumHomotopyIterations=100  PhasorMode=off  PhasorModeNumHarmonics=1  ConsistencySolver=NEWTON_XTOL_AFTER_FTOL  IndexReductionMethod=DerivativeReplacement  DoDC=off  ResidualTolerance=1e-09  ConsistencyTolSource=GLOBAL  ConsistencyAbsTol=0.001  ConsistencyRelTol=0.001  ConsistencyTolFactor=0.001  UseLocalSolver=off  LocalSolverChoice=NE_BACKWARD_EULER_ADVANCER  ResolveIndetEquations=on  FunctionEvalNumThread=1  LocalSolverSampleTime=0.001  DoFixedCost=off  MaxNonlinIter=3  MaxModeIter=2  ComputeImpulses=off  ImpulseIterations=2  LinearAlgebra=auto  LinearAlgebraNumThread=0  EquationFormulation=NE_TIME_EF  DelaysMemoryBudget=1024  AutomaticFiltering=on  FilteringTimeConstant=0.001  PartitionStorageMethod=AS_NEEDED  PartitionMemoryBudget=1024  PartitionMethod=ROBUST  MultibodyUseLocalSolver=off  MultibodyLocalSolverChoice=ODE1  MultibodyLocalSolverSampleTime=0.001
  Vds probe : fl_lib/Electrical/Electrical Sensors/Voltage Sensor
  Vds to Simulink : nesl_utility/PS-Simulink Converter  PhysicalDomain=network_engine_domain  SubClassName=ps_output  LeftPortType=input  RightPortType=output  PseudoPeriodic=off  Frequencies=[]  VectorFormat=inherit  Unit=inherit  AffineConversion=off
  Energised : Outport
  Icoil : Outport  Port=2
  Vds : Outport  Port=3
  wires:
  Icoil to Simulink/1 -> Icoil/1, Relay pulls in/1
  Relay pulls in/1 -> Energised/1
  Vds to Simulink/1 -> Vds/1
  Q/1 -> HC00 edge (1 us)/1
  HC00 edge (1 us)/1 -> Q to PS/1
  connections:
  Q to PS/RConn1 -- Gate drive/RConn1
  Gate drive/LConn1 -- Driver MOSFET/LConn1
  Gate drive/RConn2 -- GND_gate/LConn1
  Coil/LConn1 -- 5V rail/LConn1 -- Flyback diode/RConn1
  Coil/RConn1 -- Coil current/LConn1
  Coil current/RConn2 -- Driver MOSFET/RConn1 -- Flyback diode/LConn1 -- Vds probe/LConn1
  Coil current/RConn1 -- Icoil to Simulink/LConn1
  Driver MOSFET/RConn2 -- GND_src/LConn1
  GND_rail/LConn1 -- 5V rail/RConn1 -- Solver Config/RConn1
  Vds probe/RConn2 -- GND_vds/LConn1
  Vds probe/RConn1 -- Vds to Simulink/LConn1

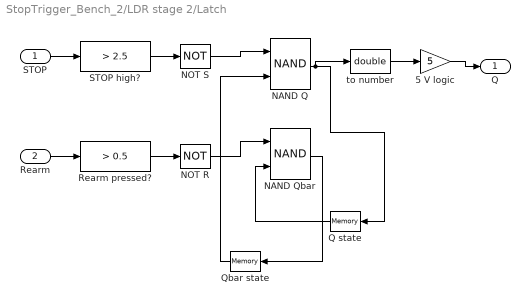
== system StopTrigger_Bench_2/LDR stage 2/Latch ==
  STOP : Inport
  Rearm : Inport  Port=2
  5 V logic : Gain  Gain=5
  NAND Q : Logic  Operator=NAND  AllPortsSameDT=off  OutDataTypeStr=boolean
  NAND Qbar : Logic  Operator=NAND  AllPortsSameDT=off  OutDataTypeStr=boolean
  NOT R : Logic  Operator=NOT  AllPortsSameDT=off  OutDataTypeStr=boolean
  NOT S : Logic  Operator=NOT  AllPortsSameDT=off  OutDataTypeStr=boolean
  Q state : Memory
  Qbar state : Memory  InitialCondition=1
  Rearm pressed? : simulink/Logic and Bit Operations/Compare To Constant  relop=>  const=0.5  OutDataTypeStr=boolean
  STOP high? : simulink/Logic and Bit Operations/Compare To Constant  relop=>  const=2.5  OutDataTypeStr=boolean
  to number : DataTypeConversion  OutDataTypeStr=double  SaturateOnIntegerOverflow=off  RndMeth=Floor
  Q : Outport
  wires:
  STOP/1 -> STOP high?/1
  STOP high?/1 -> NOT S/1
  NOT S/1 -> NAND Q/1
  Rearm/1 -> Rearm pressed?/1
  Rearm pressed?/1 -> NOT R/1
  NOT R/1 -> NAND Qbar/1
  NAND Q/1 -> Q state/1, to number/1
  Q state/1 -> NAND Qbar/2
  NAND Qbar/1 -> Qbar state/1
  Qbar state/1 -> NAND Q/2
  to number/1 -> 5 V logic/1
  5 V logic/1 -> Q/1

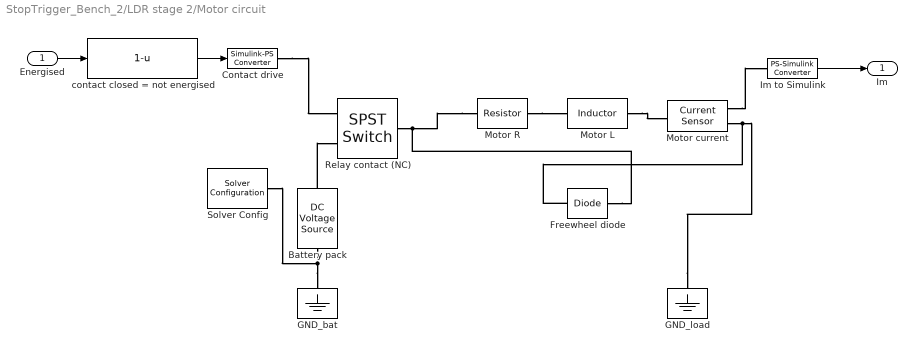
== system StopTrigger_Bench_2/LDR stage 2/Motor circuit ==
  Energised : Inport
  Battery pack : fl_lib/Electrical/Electrical Sources/DC Voltage Source  v0=2.2 V
  Contact drive : nesl_utility/Simulink-PS Converter  PhysicalDomain=network_engine_domain  SubClassName=ps_input  LeftPortType=input  RightPortType=output  PseudoPeriodic=off  Frequencies=[]  NoiseDistribution=none  NoiseParameters=[]  Unit=1  AffineConversion=off  FilteringAndDerivatives=filter  SimscapeFilterOrder=1  InputFilterTimeConstant=1e-6  UdotUserProvided=0
  Freewheel diode : ee_lib/Semiconductors & Converters/Diode  ModelType=ee.enum.diode.modelType.pwl  TableType=ee.enum.diode.tableType.IfMat  IfMat=[.07, .12, .19, 1.75, 4.24, 7.32, 11.2; .16, .3, .72, 2.14, 5.02, 8.35, 13.12] A  VfMat=[.9, 1.15, 1.25, 1.5, 1.75, 2.17, 2.6, 2.85; .58, .68, .75, 1.1, 1.38, 1.77, 2.27, 2.7] V  TjVec=[25, 125] degC  VfVec=[.5, .7, .9, 1.3, 1.7, 2.1, 2.5] V  IfVec=[.1, .2, .5, 1, 2, 4, 7, 10] A  IrMat=[1e-06, 2e-06, 5e-06, 1e-05, 2.5e-05, 5e-05, .0001; 2e-06, 5e-06, 1e-05, 4e-05, 8e-05, .0002, .0005] A  VrMat=[10, 100, 200, 250, 300, 325, 350; 10, 70, 160, 220, 270, 300, 320] V  VrVec=[10, 20, 40, 50, 70, 80, 100] V  IrVec=[1e-06, 2e-06, 5e-06, 1e-05, 2e-05, 5e-05, .0001] A  Vf=0.6 V  Ron=0.3 Ohm  Goff=1e-8 S  prmExp=ee.enum.diode.expParam.useTwo  I12=[.0137, .545] A  V12=[.6, .7] V  RS=0 Ohm  Tmeas=298.15 K  IS=1e-12 A  ec=1  I1=0.0137 A  V1=0.6 V  N_series=1  N_parallel=1  ZenerEnable=false  Rz=0.3 Ohm  BV=inf V  C_param=ee.enum.diode.capParam.fixed  CJ=0 pF  CJ0=5 pF  Vvec=[.1, 10, 100] V  Cvec=[3.5, 1, .4] pF  VJ=1 V  Mgrad=0.5  FC=0.5  Q_param=ee.enum.diode.recoveryParam.off  iRM=-7.15 A  iF=4 A  didt=-750 A/us  trr_factor=3  trr=115 ns  Qrr=150 nA*s  Vr=-600 V  Ls=150 nH  Erec=0.03 J  TT=50 ns  tau=100 ns  T_param=ee.enum.diode.temperatureParam.off  Tdevice=298.15 K  I1_T2=0.245 A  V1_T2=0.5 V  IS_T2=1.25e-7 A  Tmeas2=125 degC  XTI_param=ee.enum.diode.xtiParam.pn  XTI=3  EG_param=ee.enum.diode.egapParam.material_si  EG=1.11 eV  dBVdT=0 V/K  enable_fault_input=simscape.enum.onoff.off  i_specify=off  i_priority=None  i=0 A  i_nominal_specify=off  i_nominal_value=1  i_nominal_unit=A  v_specify=off  v_priority=None  v=0 V  v_nominal_specify=off  v_nominal_value=1  v_nominal_unit=V  v_capacitor_specify=off  v_capacitor_priority=None  v_capacitor=0 V  v_capacitor_nominal_specify=off  v_capacitor_nominal_value=1  v_capacitor_nominal_unit=V  Qj_specify=off  Qj_priority=High  Qj=0 C  Qj_nominal_specify=off  Qj_nominal_value=1  Qj_nominal_unit=C  i_diode_specify=off  i_diode_priority=None  i_diode=0 A  i_diode_nominal_specify=off  i_diode_nominal_value=1  i_diode_nominal_unit=A  v_diode_specify=off  v_diode_priority=None  v_diode=0 V  v_diode_nominal_specify=off  v_diode_nominal_value=1  v_diode_nominal_unit=V  i_capacitor_specify=off  i_capacitor_priority=None  i_capacitor=0 A  i_capacitor_nominal_specify=off  i_capacitor_nominal_value=1  i_capacitor_nominal_unit=A  power_dissipated_specify=off  power_dissipated_priority=None  power_dissipated=0 W  power_dissipated_nominal_specify=off  power_dissipated_nominal_value=1  power_dissipated_nominal_unit=W  fidelity_level=ee.enum.diode.fidelity.includeChargeDyn  rec_loss_model=ee.enum.diode.reverseRecoveryModel.fixed  ErecVal=0 J  scaleWithIandV=true  ErecMat=zeros(2, 3) J  TjrecVec=[298.15, 398.15] K  IfrecVec=[.1, 1, 10] A  IrecVal=10 A  VrecVal=10 V  tFilter=1 / 1000 / 100 s  thermal_network_parameterization=ee.enum.thermalNetworkTopology.junctionCase  Rth=[0, 10] K/W  Rth_Cauer=[1, 3, 10] K/W  Rth_Foster=[.08, .14, .22, .16] K/W  thermal_mass_parameterization=ee.enum.thermalNetwork.timeconstant  thermal_mass=[0, 1] J/K  thermal_mass_Cauer=[.1, .3, 1] J/K  thermal_mass_Foster=[.001, .005, .05, .5] J/K  thermal_time_constant=[0, 10] s  thermal_time_constant_Cauer=[1, 3, 10] s  thermal_time_constant_Foster=[7e-05, .0007, .01, .08] s  thermal_mass_initial_temperatures=[25, 25] degC  thermal_mass_initial_temperatures_Cauer=[25, 25, 25] degC  junction_thermal_mass=0.01 J/K  Tvec_initial_Foster=[25, 25, 25, 25] degC  no_thermal_network=0  junction_temperature_specify=off  junction_temperature_priority=None  junction_temperature=25 degC  junction_temperature_nominal_specify=off  junction_temperature_nominal_value=1  junction_temperature_nominal_unit=degC
  GND_bat : fl_lib/Electrical/Electrical Elements/Electrical Reference
  GND_load : fl_lib/Electrical/Electrical Elements/Electrical Reference
  Im to Simulink : nesl_utility/PS-Simulink Converter  PhysicalDomain=network_engine_domain  SubClassName=ps_output  LeftPortType=input  RightPortType=output  PseudoPeriodic=off  Frequencies=[]  VectorFormat=inherit  Unit=inherit  AffineConversion=off
  Motor L : fl_lib/Electrical/Electrical Elements/Inductor  l=2e-3 H  r=0 Ohm  g=1e-9 1/Ohm  i_specify=off  i_priority=None  i=0 A  i_nominal_specify=off  i_nominal_value=1  i_nominal_unit=A  v_specify=off  v_priority=None  v=0 V  v_nominal_specify=off  v_nominal_value=1  v_nominal_unit=V  i_L_specify=off  i_L_priority=High  i_L=0 A  i_L_nominal_specify=off  i_L_nominal_value=1  i_L_nominal_unit=A
  Motor R : fl_lib/Electrical/Electrical Elements/Resistor  R=4.5 Ohm  i_specify=off  i_priority=None  i=0 A  i_nominal_specify=off  i_nominal_value=1  i_nominal_unit=A  v_specify=off  v_priority=None  v=0 V  v_nominal_specify=off  v_nominal_value=1  v_nominal_unit=V
  Motor current : fl_lib/Electrical/Electrical Sensors/Current Sensor
  Relay contact (NC) : ee_lib/Switches & Breakers/SPST Switch  R_closed=0.05 Ohm  G_open=1e-9 S  Threshold=0.5 V  Width=0 V  model_dynamics=1  t_on=3e-3 s  t_off=8e-3 s  initial_vT=0 V
      settings: InternalSimscapePortConfiguration="{\"Bottom\":[],\"Left\":[{\"id\":\"vT\",\"label\":\"vT\",\"type\":\"input\"},{\"id\":\"p\",\"label\":\"\",\"type\":\"foundation.electrical.electrical\"}],\"Right\":[{\"id\":\"n\",\"label\":\"\",\"type\":\"foundation.electrical.electrical\"}],\"Top\":[]}"
  Solver Config : nesl_utility/Solver Configuration  PhysicalDomain=network_engine_domain  SubClassName=solver  LeftPortType=input  RightPortType=generic  Tones=[]  Harmonics=[]  SimulateNoise=off  Profile=off  UseLocalSampling=off  EnableSwitchedLinearOptims=on  FrequencyDomain=off  UseCCode=off  RelTol=0.001  AbsTol=0.001  MinStep=1e-09  ToWorkspace=off  RevertToSquareIcSolve=off  NumHomotopyIterations=100  PhasorMode=off  PhasorModeNumHarmonics=1  ConsistencySolver=NEWTON_XTOL_AFTER_FTOL  IndexReductionMethod=DerivativeReplacement  DoDC=off  ResidualTolerance=1e-09  ConsistencyTolSource=GLOBAL  ConsistencyAbsTol=0.001  ConsistencyRelTol=0.001  ConsistencyTolFactor=0.001  UseLocalSolver=off  LocalSolverChoice=NE_BACKWARD_EULER_ADVANCER  ResolveIndetEquations=on  FunctionEvalNumThread=1  LocalSolverSampleTime=0.001  DoFixedCost=off  MaxNonlinIter=3  MaxModeIter=2  ComputeImpulses=off  ImpulseIterations=2  LinearAlgebra=auto  LinearAlgebraNumThread=0  EquationFormulation=NE_TIME_EF  DelaysMemoryBudget=1024  AutomaticFiltering=on  FilteringTimeConstant=0.001  PartitionStorageMethod=AS_NEEDED  PartitionMemoryBudget=1024  PartitionMethod=ROBUST  MultibodyUseLocalSolver=off  MultibodyLocalSolverChoice=ODE1  MultibodyLocalSolverSampleTime=0.001
  contact closed = not energised : Fcn  Expr=1-u
  Im : Outport
  wires:
  Energised/1 -> contact closed = not energised/1
  contact closed = not energised/1 -> Contact drive/1
  Im to Simulink/1 -> Im/1
  connections:
  Contact drive/RConn1 -- Relay contact (NC)/LConn1
  Battery pack/LConn1 -- Relay contact (NC)/LConn2
  Motor R/LConn1 -- Relay contact (NC)/RConn1 -- Freewheel diode/RConn1
  Motor R/RConn1 -- Motor L/LConn1
  Motor L/RConn1 -- Motor current/LConn1
  GND_load/LConn1 -- Motor current/RConn2 -- Freewheel diode/LConn1
  Motor current/RConn1 -- Im to Simulink/LConn1
  GND_bat/LConn1 -- Battery pack/RConn1 -- Solver Config/RConn1
